simulink model "golden_mnist_q8_v1"  (R2026b)
settings: Solver=FixedStepAuto
model workspace (MAT data in the model file):
  qNet : dlnetwork (value not decoded)
symbols that are objects in the model workspace (value not decoded): qNet
libraries: dlconvfclib x3, dlactivationlib x3, dlinputlayernormlib x1, dlpoolinglib x1
settings Model: Creator=hkawai  LastModifiedBy=hkawai
settings OptimizationCC: DefaultParameterBehavior=Inlined  DifferentSizesBufferReuse=on  EfficientTunableParamExpr=on  EnhancedBackFolding=on  OptimizationCustomize=off  OptimizeBlockOrder=speed  PassReuseOutputArgsAs=Individual arguments  RemoveInternalMemoryZeroInit=on  RemoveRootLevelIOMemoryZeroInit=on
settings DebuggingCC: ParameterTunabilityLossMsg=error
settings SFSimCC: MATLABDynamicMemAlloc=off
settings RTWCC: DataTypeReplacement=CDataTypesFixedWidth  Description=Embedded Coder  SystemTargetFile=ert.tlc  TemplateMakefile=ert_default_tmf
settings CodeAppCC: ForceParamTrailComments=on  IgnoreCustomStorageClasses=off  InsertBlockDesc=on  OperatorAnnotations=on  SFDataObjDesc=on  SimulinkDataObjDesc=on
settings ERTTargetCC: CombineSignalStateStructs=on  GenerateSampleERTMain=on  MaxIdInt16=INT16_MAX  MaxIdInt32=INT32_MAX  MaxIdInt64=INT64_MAX  MaxIdInt8=INT8_MAX  MaxIdUint16=UINT16_MAX  MaxIdUint32=UINT32_MAX  MaxIdUint64=UINT64_MAX  MaxIdUint8=UINT8_MAX  MinIdInt16=INT16_MIN  MinIdInt32=INT32_MIN  MinIdInt64=INT64_MIN  MinIdInt8=INT8_MIN

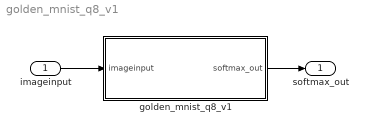
== system golden_mnist_q8_v1 ==
  imageinput : Inport  PortDimensions="[28  28   1]"  SampleTime=1
  golden_mnist_q8_v1 : Subsystem
  softmax_out : Outport
  wires:
  imageinput/1 -> golden_mnist_q8_v1/1(imageinput)
  golden_mnist_q8_v1/1(softmax_out) -> softmax_out/1

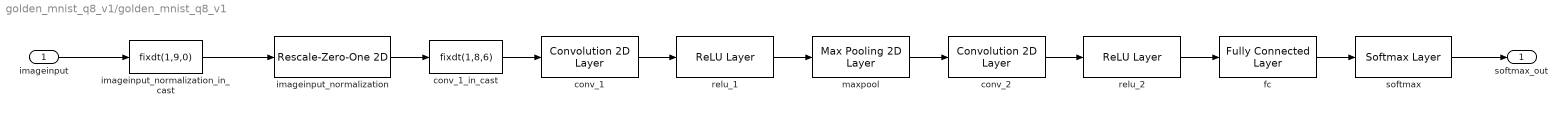
== system golden_mnist_q8_v1/golden_mnist_q8_v1 ==
  imageinput : Inport  PortDimensions="[28  28   1]"  SampleTime=1
  conv_1 : dlconvfclib/Convolution 2D Layer  Layer=qNet.Layers(2)  OutMin=[]  OutMax=[]  OutDataTypeStr=fixdt(1,8,5)  RndMeth=Nearest  SaturateOnIntegerOverflow=on  WeightsDataTypeStr=fixdt(1,8,6)  WeightsMin=[]  WeightsMax=[]  BiasDataTypeStr=fixdt(1,32,12)  BiasMin=[]  BiasMax=[]  AccumDataTypeStr=fixdt(1,32,12)  InternalRndMeth=Nearest  InternalSaturateOnIntegerOverflow=off  SampleTime=1
      settings: DataFormat=SSC
  conv_1_in_cast : DataTypeConversion  OutDataTypeStr=fixdt(1,8,6)  RndMeth=Nearest
  conv_2 : dlconvfclib/Convolution 2D Layer  Layer=qNet.Layers(5)  OutMin=[]  OutMax=[]  OutDataTypeStr=fixdt(1,8,4)  RndMeth=Nearest  SaturateOnIntegerOverflow=on  WeightsDataTypeStr=fixdt(1,8,6)  WeightsMin=[]  WeightsMax=[]  BiasDataTypeStr=fixdt(1,32,11)  BiasMin=[]  BiasMax=[]  AccumDataTypeStr=fixdt(1,32,11)  InternalRndMeth=Nearest  InternalSaturateOnIntegerOverflow=off  SampleTime=1
      settings: DataFormat=SSC
  fc : dlconvfclib/Fully Connected Layer  Layer=qNet.Layers(7)  InputSize=1  OutMin=[]  OutMax=[]  OutDataTypeStr=fixdt(1,8,1)  RndMeth=Nearest  SaturateOnIntegerOverflow=on  WeightsDataTypeStr=fixdt(1,8,6)  WeightsMin=[]  WeightsMax=[]  BiasDataTypeStr=fixdt(1,32,10)  BiasMin=[]  BiasMax=[]  AccumDataTypeStr=fixdt(1,32,10)  AccumMin=[]  AccumMax=[]  InternalRndMeth=Nearest  InternalSaturateOnIntegerOverflow=off  SampleTime=1
      settings: DataFormat=SSC
  imageinput_normalization : dlinputlayernormlib/Rescale-Zero-One 2D  Layer=qNet.Layers(1)  OutMin=[]  OutMax=[]  OutDataTypeStr=fixdt(0,8,8)  RndMeth=Nearest  SaturateOnIntegerOverflow=on  MinDataTypeStr=fixdt(0,8,0)  MinMin=[]  MinMax=[]  MaxDataTypeStr=fixdt(0,8,0)  MaxMin=[]  MaxMax=[]  DivideOutDataTypeStr=fixdt(0,8,8)  DivideOutMin=[]  DivideOutMax=[]  SubtractMinAccumDataTypeStr=fixdt(1,9,0)  InternalRndMeth=Nearest  InternalSaturateOnIntegerOverflow=on  SampleTime=1
      settings: DataFormat=SSC
  imageinput_normalization_in_cast : DataTypeConversion  OutDataTypeStr=fixdt(1,9,0)  RndMeth=Nearest
  maxpool : dlpoolinglib/Max Pooling 2D Layer  Layer=qNet.Layers(4)  OutMin=[]  OutMax=[]  OutDataTypeStr=fixdt(1,8,5)  SampleTime=1
      settings: DataFormat=SSC
  relu_1 : dlactivationlib/ReLU Layer  OutMin=[]  OutMax=[]  OutDataTypeStr=fixdt(1,8,5)  SampleTime=1
  relu_2 : dlactivationlib/ReLU Layer  OutMin=[]  OutMax=[]  OutDataTypeStr=fixdt(1,8,4)  SampleTime=1
  softmax : dlactivationlib/Softmax Layer  ApproximationMethod=Lookup  OutMin=[]  OutMax=[]  OutDataTypeStr=fixdt(0,8,8)  RndMeth=Nearest  SaturateOnIntegerOverflow=on  AccumDataTypeStr=fixdt(0,32,16)  InternalRndMeth=Nearest  InternalSaturateOnIntegerOverflow=on  SampleTime=1
      settings: DataFormat=C
  softmax_out : Outport
  wires:
  imageinput_normalization/1 -> conv_1_in_cast/1
  imageinput/1 -> imageinput_normalization_in_cast/1
  imageinput_normalization_in_cast/1 -> imageinput_normalization/1
  softmax/1 -> softmax_out/1
  conv_1_in_cast/1 -> conv_1/1
  maxpool/1 -> conv_2/1
  conv_2/1 -> relu_2/1
  relu_1/1 -> maxpool/1
  conv_1/1 -> relu_1/1
  relu_2/1 -> fc/1
  fc/1 -> softmax/1
